simulink model "Working_with_RLC_3"  (R2024a)
settings: Solver=ode4  StartTime=0.0  StopTime=0.1  FixedStep=1e-4  RelTol=1e-3
libraries: mpclib x1, slpidlib x1
settings Model: Creator=anshu  LastModifiedBy=anshu

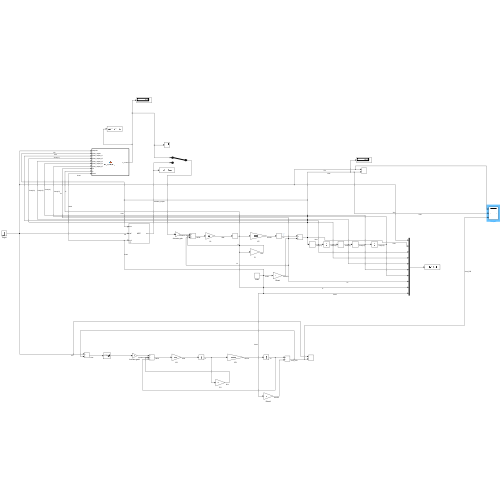
[thumbnail: Simulink's stored preview of the top-level diagram]
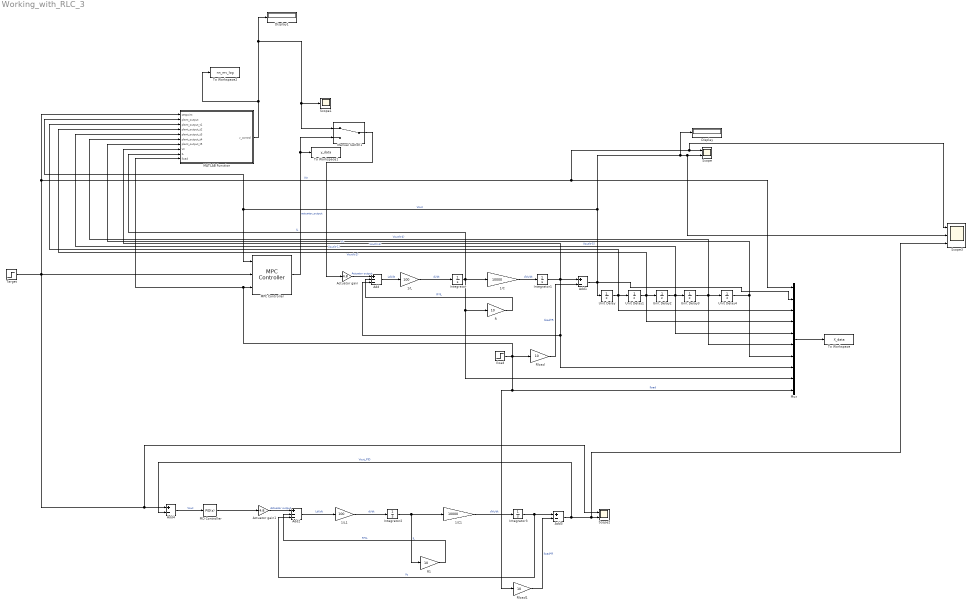
== system Working_with_RLC_3 ==
  1/C : Gain  Gain=10000
  1/C1 : Gain  Gain=10000
  1/L : Gain  Gain=100
  1/L1 : Gain  Gain=100
  Actuator gain : Gain  Gain=4.8
  Actuator gain1 : Gain  Gain=4.8
  Add : Sum  Inputs=+--
  Add1 : Sum  Inputs=+-
  Add2 : Sum  Inputs=+--
  Add3 : Sum  Inputs=+-
  Add4 : Sum  Inputs=+-
  Display : Display
  Display1 : Display
  Iload : Step  Time=0.04  After=0.3  SampleTime=1e-4
  Integrator{,1..3} (4 alike) : Integrator
  MATLAB Function : MATLAB Function  TreatAsAtomicUnit=on
  MPC Controller : mpclib/MPC Controller  SCDEnableBlockLinearizationSpecification=on  mpcobj=mpc_controller_3  x0=mpc_initial_state_3  is_multiple=0  enable_value=0  return_u0=off  updateMPCinCallerWorkspace=on  md_inport=on  mv_inport=off  uref_inport=off  return_cost=off  return_mvseq=off  return_qpstatus=off  return_xseq=off  return_state=off  return_ovseq=off  state_inport=off  umin_inport=off  umax_inport=off  ymin_inport=off  ymax_inport=off  cc_inport=off  ywt_inport=off  uwt_inport=off  duwt_inport=off  rhoeps_inport=off  pm_inport=off  MaximumP=10  HorizonChoice=FixedHorizon  n_ts=0.0001  n_p=50  n_mv=1  n_md=1  n_ud=0  n_mo=1  n_uo=0  BlockDataType=double  SampleTimeInherited=off  switch_inport=off
  Manual Switch1 : ManualSwitch
  Mux : Mux  Inputs=10
  PID Controller : slpidlib/PID Controller  Controller=PID  Form=Parallel  TimeDomain=Continuous-time  UseExternalTs=off  SampleTime=-1  IntegratorMethod=Forward Euler  FilterMethod=Forward Euler  ControllerParametersSource=internal  P=0.434968116146811  I=247.914401992375  UseKiTs=off  D=0.000189556773354288  UseExternalDerivativeSource=off  N=100  UseFilter=on  TunerSelectOption=Transfer Function Based (PID Tuner App)  InitialConditionSource=internal  InitialConditionForIntegrator=0  InitialConditionForFilter=0  DifferentiatorICPrevScaledInput=0  ExternalReset=none  TrackingMode=off  Kt=1  LimitOutput=on  SatLimitsSource=internal  UpperSaturationLimit=5  LowerSaturationLimit=0  LinearizeAsGain=on  AntiWindupMode=none  Kb=1  LimitIntegrator=off  UpperIntegratorSaturationLimit=inf  LowerIntegratorSaturationLimit=-inf  POutMin=[]  POutMax=[]  IOutMin=[]  IOutMax=[]  DOutMin=[]  DOutMax=[]  NOutMin=[]  NOutMax=[]  SumOutMin=[]  SumOutMax=[]  SaturationOutMin=[]  SaturationOutMax=[]  PParamMin=[]  PParamMax=[]  IParamMin=[]  IParamMax=[]  DParamMin=[]  DParamMax=[]  NParamMin=[]  NParamMax=[]  KbParamMin=[]  KbParamMax=[]  KtParamMin=[]  KtParamMax=[]  KbOutMin=[]  KbOutMax=[]  KtOutMin=[]  KtOutMax=[]  IntegratorOutMin=[]  IntegratorOutMax=[]  FilterOutMin=[]  FilterOutMax=[]  SumI1OutMin=[]  SumI1OutMax=[]  SumI2OutMin=[]  SumI2OutMax=[]  SumI3OutMin=[]  SumI3OutMax=[]  SumI4OutMin=[]  SumI4OutMax=[]  SumDOutMin=[]  SumDOutMax=[]  DifferentiatorOutMin=[]  DifferentiatorOutMax=[]  FilterDiffOutCoefMin=[]  FilterDiffOutCoefMax=[]  ReciprocalOutMin=[]  ReciprocalOutMax=[]  SumDenOutMin=[]  SumDenOutMax=[]  SumNumOutMin=[]  SumNumOutMax=[]  DivideOutMin=[]  DivideOutMax=[]  UdiffTsProdOutMin=[]  UdiffTsProdOutMax=[]  NTsProdOutMin=[]  NTsProdOutMax=[]  UintegralTsProdOutMin=[]  UintegralTsProdOutMax=[]  UngainTsProdOutMin=[]  UngainTsProdOutMax=[]  ClampingZeroOutDataTypeStr=Inherit: Inherit via back propagation  ClampingZeroOutMin=[]  ClampingZeroOutMax=[]  FilterDenConstantOutDataTypeStr=Inherit: Inherit via back propagation  FilterDenConstantOutMin=[]  FilterDenConstantOutMax=[]  PCopyOutDataTypeStr=Inherit: Inherit via back propagation  PCopyOutMin=[]  PCopyOutMax=[]  NCopyOutDataTypeStr=Inherit: Inherit via back propagation  NCopyOutMin=[]  NCopyOutMax=[]  IntegratorContinuousStateAttributes=''  IntegratorStateMustResolveToSignalObject=off  IntegratorRTWStateStorageClass=Auto  FilterContinuousStateAttributes=''  FilterStateMustResolveToSignalObject=off  FilterRTWStateStorageClass=Auto  ParallelPVariant=InternalParameters  IdealPVariant=Disabled  IVariant=InternalParameters  DVariant=InternalParameters  IntegratorVariant=Continuous  SatVariant=Enabled  AWVariant=Passthrough  PCopyVariant=Disabled  TRVariant=Disabled  FdbkBlocksVariant=Forward  IdealPFdbkVariant=Disabled  SatFdbkVariant=Disabled  DerivativeFilterVariant=ContFilter  NVariant=InternalParameters  NCopyVariant=Disabled  FilterICVariant=InternalICsFilter  IntegratorICVariant=InternalICs  ExternalResetVariant=Disabled  TRSumVariant=Passthrough  SumFdbkVariant=Disabled  SumVariant=Sum_PID  TsampFilterVariant=InternalTs  TsampNgainVariant=Passthrough  TsampIntegralVariant=Disabled_SignalSpec  ExternalSaturationOutDataTypeStr=Inherit: Same as second input  DerivativeSourceVariant=ErrorSignal
  R : Gain  Gain=10
  R1 : Gain  Gain=10
  Rload : Gain  Gain=10
  Rload1 : Gain  Gain=10
  Scope : Scope  NumInputPorts=2
  Scope1 : Scope
  Scope2 : Scope  NumInputPorts=2
  Scope3 : Scope  NumInputPorts=3
  Target : Step  Time=0.01  After=19  SampleTime=1e-4
  To Workspace : ToWorkspace  VariableName=X_data  SampleTime=-1
      settings: Save2DSignal=2-D array (concatenate along first dimension)
  To Workspace1 : ToWorkspace  VariableName=y_data  SampleTime=-1
      settings: Save2DSignal=2-D array (concatenate along first dimension)
  To Workspace2 : ToWorkspace  VariableName=nn_mv_log  SampleTime=-1
  Unit Delay{,1..4} (5 alike) : UnitDelay  SampleTime=0.0001  HasFrameUpgradeWarning=on
  wires:
  Add/1 -> 1/L/1  "Ldi/dt"
  1/L/1 -> Integrator/1  "di/dt"
  Integrator/1 -> MATLAB Function/9(IL), 1/C/1, Mux/9, R/1  "IL"
  Iload/1 -> Rload/1, Mux/10, Rload1/1, MATLAB Function/10(Iload), MPC Controller/3  "Iload"
  R/1 -> Add/2  "R*IL"
  1/C/1 -> Integrator1/1  "dVc/dt"
  Integrator1/1 -> MATLAB Function/8(Vc), Mux/8, Add/3, Add1/1  "Vc"
  Rload/1 -> Add1/2  "Iload*R"
  Add1/1 -> Display/1, Scope3/2, Scope/2, MATLAB Function/2(plant_output), MPC Controller/1, Unit Delay/1, Mux/2  "Vout"
  MPC Controller/1 -> Manual Switch1/2, To Workspace1/1  "actuator_output"
  Unit Delay/1 -> MATLAB Function/3(plant_output_t1), Mux/3, Unit Delay1/1  "Vout(t-1)"
  Unit Delay1/1 -> MATLAB Function/4(plant_output_t2), Mux/4, Unit Delay2/1  "Vout(t-2)"
  Unit Delay2/1 -> MATLAB Function/5(plant_output_t3), Mux/5, Unit Delay3/1  "Vout(t-3)"
  Unit Delay3/1 -> MATLAB Function/6(plant_output_t4), Mux/6, Unit Delay4/1  "Vout(t-4)"
  Unit Delay4/1 -> MATLAB Function/7(plant_output_t5), Mux/7  "Vout(t-5)"
  Mux/1 -> To Workspace/1
  Actuator gain/1 -> Add/1  "Actuator output"
  Manual Switch1/1 -> Actuator gain/1
  MATLAB Function/1(v_control) -> To Workspace2/1, Display1/1, Manual Switch1/1, Scope1/1
  1/L1/1 -> Integrator2/1  "di/dt"
  Integrator2/1 -> R1/1, 1/C1/1  "IL"
  1/C1/1 -> Integrator3/1  "dVc/dt"
  Add2/1 -> 1/L1/1  "Ldi/dt"
  Actuator gain1/1 -> Add2/1  "Actuator output"
  Integrator3/1 -> Add2/3, Add3/1  "Vc"
  Rload1/1 -> Add3/2  "Iload*R"
  R1/1 -> Add2/2  "R*IL"
  PID Controller/1 -> Actuator gain1/1
  Target/1 -> MPC Controller/2, Scope3/1, Scope/1, Mux/1, MATLAB Function/1(setpoint), Scope2/1, Add4/1  "Vin"
  Add4/1 -> PID Controller/1  "Vout"
  Add3/1 -> Scope3/3, Scope2/2, Add4/2  "Vout_PID"

== matlab function Working_with_RLC_3/MATLAB Function ==
  data: setpoint input; v_control output; plant_output input; plant_output_t1 input; plant_output_t2 input; plant_output_t3 input; plant_output_t4 input; plant_output_t5 input; Vc input; IL input; Iload input
function v_control = nn_controller_3(setpoint, plant_output, plant_output_t1,...
                                     plant_output_t2, plant_output_t3, ...
                                     plant_output_t4, plant_output_t5, ...
                                     Vc, IL, Iload)
%% Function block to import the weights and biases of a trained neural network
%   The exported weights are to be taken from nn_weights_for_matlab_3.mat
%   The inputs have to be passed in exactly the same order (Must match the
%   list Features as generated in Python....
%   i.e., Vin, Vout, Vout (t-1)...Vout(t-5), Vc, IL, Iload

%% Define the required variables for the function as persistent...
persistent W1 W2 W3 W4 W5 W6 b1 b2 b3 b4 b5 b6 act1 act2 act3 act4 act5 act6 ...
           input_mean input_std ...
           output_mean output_std U_min U_max num_layers

%% 1. Load the required data
if isempty(num_layers)
    % load the nn weights from matlab
    loaded_data = coder.load('nn_weights_for_matlab_3.mat');
    num_layers = 6;
    
    
    W1 = loaded_data.W1; b1 = loaded_data.b1; act1 = char(loaded_data.activation1);
    W2 = loaded_data.W2; b2 = loaded_data.b2; act2 = char(loaded_data.activation2);
    W3 = loaded_data.W3; b3 = loaded_data.b3; act3 = char(loaded_data.activation3);
    W4 = loaded_data.W4; b4 = loaded_data.b4; act4 = char(loaded_data.activation4);
    W5 = loaded_data.W5; b5 = loaded_data.b5; act5 = char(loaded_data.activation5);
    W6 = loaded_data.W6; b6 = loaded_data.b6; act6 = char(loaded_data.activation6);
    input_mean = loaded_data.input_mean;
    input_std = loaded_data.input_std;
    output_mean = loaded_data.output_mean;
    output_std = loaded_data.output_std;
    U_min = loaded_data.u_min;
    U_max = loaded_data.u_max;

end
%% 2. Assemble the input row vector in the exact training order
features = [setpoint, plant_output, plant_output_t1, ...
            plant_output_t2, plant_output_t3, ...
            plant_output_t4, plant_output_t5, ...
            Vc, IL, Iload];

%%% 2.1. Normalize in the same way as normalization was done during
%%% training
features_norm = (features - input_mean) ./ input_std;

%% 3. The forward pass....
h1 = features_norm * W1 + b1;
if strcmp(act1, 'relu'), h1 = max(h1, 0);
elseif ~strcmp(act1, 'linear'), error('Unsupported activation: %s', act1');
end

h2 = h1 * W2 + b2;
if strcmp(act2, 'relu'), h2 = max(h2, 0);
elseif ~strcmp(act2, 'linear'), error('Unsupported activation: %s', act2');
end

h3 = h2 * W3 + b3;
if strcmp(act3, 'relu'), h3 = max(h3, 0);
elseif ~strcmp(act3, 'linear'), error('Unsupported activation: %s', act3');
end

h4 = h3 * W4 + b4;
if strcmp(act4, 'relu'), h4 = max(h4, 0);
elseif ~strcmp(act4, 'linear'), error('Unsupported activation: %s', act4);
end

h5 = h4 * W5 + b5;
if strcmp(act5, 'relu'), h5 = max(h5, 0);
elseif ~strcmp(act5, 'linear'), error('Unsupported activation: %s', act5);
end

out = h5 * W6 + b6;
if strcmp(act6, 'relu'), out = max(out, 0);
elseif ~strcmp(act6, 'linear'), error('Unsupported activation: %s', act6);
end

v_control_raw = out * output_std + output_mean;

%% Zero-setpoint safety check
if features(1) < 0.1
    v_control_raw = 0.0;
    v_control = v_control_raw;
    return;
end

%% De-normalize the output and then clip it to the actuator range...
v_control = min(max(v_control_raw, U_min), U_max);

end
